simulink model "viikate_rocket"  (R2026b)
settings: Solver=ode4  StopTime=inf  FixedStep=0.001
undefined symbols (not defined in the file or in its folder): Aero, e0_0, e1_0, e2_0, e3_0, gravity, I, N, Newton, Raphson, rho, rp_burn_time_s, rp_canard_area_m2, rp_canard_cl_alpha, rp_cd0, rp_clp, rp_cmq, rp_cn_alpha, rp_cnr, rp_fin_positions_m, rp_frontal_area_m2, rp_gust_seed, rp_gust_variance, rp_ignition_time_s, rp_inertia_empty_kgm2, rp_inertia_full_kgm2, rp_length_m, rp_mass_fuel_kg, rp_mass_full_kg, rp_r_cp_m, rp_roll_ref_length_m, rp_servo_rate_limit_radps, rp_servo_tau_s, rp_thrust_n, rp_thrust_scale, rp_thrust_t_s, rp_wind_model_mps, sharedaeroassertmsg, si, Vsafe, ZYX
libraries: matrix_library x1
(part 2 of 3)

== system viikate_rocket/Simple Variable Mass 6DOF/Determine Force, Mass & Inertia/Estimate Inertia Tensor ==
  Mass : Inport
  M_dot : Inport  Port=2
  Constant : Constant  Value=emass
  Constant1 : Constant  Value=fmass
  "Interpolate Inertia " : Subsystem  mask(ScheduleMatrix-1D){matrix=I, aMode=aMode}
      mask prompts: matrix "shared_aeroblks:sharedaeroblkschedule:blockScheduleMatrix1DParamMatrixtointerpolate"
      mask help: shared_aeroblks:sharedaeroblkschedule:blockScheduleMatrix1DDesc
      mask init:
      | if aerosharedtest(gcb)
      |     aerosharedicon('shared');
      | else
      |     sharedautoicon('shared');
      | end
      mask Help: eval('if license(''test'',''Aerospace_Blockset'')aerosharedhelp(''interpolate_matrix_x'');elseif license(''test'',''Powertrain_Blockset'')sharedautohelp(''interpolate_matrix_x'');end')
      mask DialogControl matrix Prompt: Matrix to interpolate:
      mask Display:
      | port_label('input', 1,'x_k');
      | port_label('input', 2,'x_f');
      | port_label('output',1,'Matrix(x)');
  Mux : Mux  Inputs=2
  PreLook-Up Index Search : PreLookup  BreakpointsDataSource=Input port  BreakpointsData=[emass fmass]  BeginIndexSearchUsingPreviousIndexResult=on  IndexDataTypeStr=int32
      settings: InputPortMap=u0,p1
  Product : Product  SaturateOnIntegerOverflow=on  OutDataTypeStr=Inherit: Same as first input
  slope : Constant  Value=(fI - eI)/(fmass - emass)  OutDataTypeStr=Inherit: Inherit via back propagation
  Inertia : Outport  VectorParamsAs1DForOutWhenUnconnected=off
  I_dot : Outport  Port=2  VectorParamsAs1DForOutWhenUnconnected=off
  wires:
  "Interpolate Inertia "/1(Matrix(x)) -> Inertia/1
  Constant1/1 -> Mux/2
  Constant/1 -> Mux/1
  Mux/1 -> PreLook-Up Index Search/2
  PreLook-Up Index Search/1 -> "Interpolate Inertia "/1(x_k)
  PreLook-Up Index Search/2 -> "Interpolate Inertia "/2(x_f)
  Mass/1 -> PreLook-Up Index Search/1
  Product/1 -> I_dot/1
  M_dot/1 -> Product/2
  slope/1 -> Product/1

== system viikate_rocket/Simple Variable Mass 6DOF/Vbxw/Subsystem ==
  A : Inport
  B : Inport  Port=2
  Demux : Demux  Outputs=3
  Demux1 : Demux  Outputs=3
  Mux : Mux  Inputs=3
  i x j : Product  InputSameDT=on  SaturateOnIntegerOverflow=on  OutDataTypeStr=Inherit: Same as first input
  j x k : Product  InputSameDT=on  SaturateOnIntegerOverflow=on  OutDataTypeStr=Inherit: Same as first input
  k x i : Product  InputSameDT=on  SaturateOnIntegerOverflow=on  OutDataTypeStr=Inherit: Same as first input
  Out1 : Outport  VectorParamsAs1DForOutWhenUnconnected=off
  wires:
  Demux1/3 -> j x k/2
  Demux/2 -> j x k/1
  Demux/3 -> k x i/1
  Demux1/1 -> k x i/2
  Demux1/2 -> i x j/2
  Demux/1 -> i x j/1
  i x j/1 -> Mux/3
  k x i/1 -> Mux/2
  j x k/1 -> Mux/1
  B/1 -> Demux1/1
  A/1 -> Demux/1
  Mux/1 -> Out1/1

== system viikate_rocket/Simple Variable Mass 6DOF/Vbxw/Subsystem1 ==
  A : Inport
  B : Inport  Port=2
  Demux : Demux  Outputs=3
  Demux1 : Demux  Outputs=3
  Mux : Mux  Inputs=3
  i x k : Product  InputSameDT=on  SaturateOnIntegerOverflow=on  OutDataTypeStr=Inherit: Same as first input
  j x i : Product  InputSameDT=on  SaturateOnIntegerOverflow=on  OutDataTypeStr=Inherit: Same as first input
  k x j : Product  InputSameDT=on  SaturateOnIntegerOverflow=on  OutDataTypeStr=Inherit: Same as first input
  Out1 : Outport  VectorParamsAs1DForOutWhenUnconnected=off
  wires:
  j x i/1 -> Mux/3
  i x k/1 -> Mux/2
  k x j/1 -> Mux/1
  Mux/1 -> Out1/1
  Demux1/1 -> j x i/2
  Demux/2 -> j x i/1
  Demux1/3 -> i x k/2
  Demux/1 -> i x k/1
  Demux1/2 -> k x j/2
  Demux/3 -> k x j/1
  B/1 -> Demux1/1
  A/1 -> Demux/1

== system viikate_rocket/Simple Variable Mass 6DOF/Calculate DCM & Euler Angles/Quaternions to Direction Cosine Matrix/A11 ==
  normal(q) : Inport
  Demux : Demux
  Product{,1..3} (4 alike) : Product  RndMeth=Zero
  Sum : Sum  Inputs=++--
  A11 : Outport  VectorParamsAs1DForOutWhenUnconnected=off
  wires:
  Sum/1 -> A11/1
  Demux/4 -> Product/2, Product/1
  Demux/3 -> Product1/2, Product1/1
  Demux/2 -> Product2/2, Product2/1
  Demux/1 -> Product3/2, Product3/1
  Product3/1 -> Sum/1
  Product2/1 -> Sum/2
  Product1/1 -> Sum/3
  Product/1 -> Sum/4
  normal(q)/1 -> Demux/1

== system viikate_rocket/Simple Variable Mass 6DOF/Calculate DCM & Euler Angles/Quaternions to Direction Cosine Matrix/A12 ==
  normal(q) : Inport
  Demux : Demux
  Gain : Gain  Gain=2
  Product2 : Product  RndMeth=Zero
  Product3 : Product  RndMeth=Zero
  Sum : Sum  Inputs=|++
  A12 : Outport  VectorParamsAs1DForOutWhenUnconnected=off
  wires:
  Product2/1 -> Sum/2
  Product3/1 -> Sum/1
  Sum/1 -> Gain/1
  Demux/1 -> Product3/2
  Demux/2 -> Product2/1
  Demux/4 -> Product3/1
  Demux/3 -> Product2/2
  normal(q)/1 -> Demux/1
  Gain/1 -> A12/1

== system viikate_rocket/Simple Variable Mass 6DOF/Calculate DCM & Euler Angles/Quaternions to Direction Cosine Matrix/A13 ==
  normal(q) : Inport
  Demux : Demux
  Gain : Gain  Gain=2
  Product1 : Product  RndMeth=Zero
  Product2 : Product  RndMeth=Zero
  Sum : Sum  Inputs=|-+
  A13 : Outport  VectorParamsAs1DForOutWhenUnconnected=off
  wires:
  Demux/1 -> Product1/1
  Product1/1 -> Sum/1
  Product2/1 -> Sum/2
  Demux/4 -> Product2/2
  Demux/2 -> Product2/1
  Demux/3 -> Product1/2
  normal(q)/1 -> Demux/1
  Gain/1 -> A13/1
  Sum/1 -> Gain/1

== system viikate_rocket/Simple Variable Mass 6DOF/Calculate DCM & Euler Angles/Quaternions to Direction Cosine Matrix/A21 ==
  normal(q) : Inport
  Demux : Demux
  Gain : Gain  Gain=2
  Product2 : Product  RndMeth=Zero
  Product3 : Product  RndMeth=Zero
  Sum : Sum  Inputs=|-+
  A21 : Outport  VectorParamsAs1DForOutWhenUnconnected=off
  wires:
  Gain/1 -> A21/1
  normal(q)/1 -> Demux/1
  Demux/3 -> Product2/2
  Demux/4 -> Product3/1
  Demux/2 -> Product2/1
  Demux/1 -> Product3/2
  Sum/1 -> Gain/1
  Product3/1 -> Sum/1
  Product2/1 -> Sum/2

== system viikate_rocket/Simple Variable Mass 6DOF/Calculate DCM & Euler Angles/Quaternions to Direction Cosine Matrix/A22 ==
  normal(q) : Inport
  Demux : Demux
  Product{,1..3} (4 alike) : Product  RndMeth=Zero
  Sum : Sum  Inputs=+-+-
  A22 : Outport  VectorParamsAs1DForOutWhenUnconnected=off
  wires:
  normal(q)/1 -> Demux/1
  Product/1 -> Sum/4
  Product1/1 -> Sum/3
  Product2/1 -> Sum/2
  Product3/1 -> Sum/1
  Demux/1 -> Product3/1, Product3/2
  Demux/2 -> Product2/1, Product2/2
  Demux/3 -> Product1/1, Product1/2
  Demux/4 -> Product/1, Product/2
  Sum/1 -> A22/1

== system viikate_rocket/Simple Variable Mass 6DOF/Calculate DCM & Euler Angles/Quaternions to Direction Cosine Matrix/A23 ==
  normal(q) : Inport
  Demux : Demux
  Gain : Gain  Gain=2
  Product1 : Product  RndMeth=Zero
  Product2 : Product  RndMeth=Zero
  Sum : Sum  Inputs=|++
  A23 : Outport  VectorParamsAs1DForOutWhenUnconnected=off
  wires:
  Demux/4 -> Product2/2
  Product2/1 -> Sum/2
  Product1/1 -> Sum/1
  Sum/1 -> Gain/1
  Demux/1 -> Product1/1
  Demux/2 -> Product1/2
  Demux/3 -> Product2/1
  Gain/1 -> A23/1
  normal(q)/1 -> Demux/1

== system viikate_rocket/Simple Variable Mass 6DOF/Calculate DCM & Euler Angles/Quaternions to Direction Cosine Matrix/A31 ==
  normal(q) : Inport
  Demux : Demux
  Gain : Gain  Gain=2
  Product1 : Product  RndMeth=Zero
  Product2 : Product  RndMeth=Zero
  Sum : Sum  Inputs=|++
  A31 : Outport  VectorParamsAs1DForOutWhenUnconnected=off
  wires:
  Sum/1 -> Gain/1
  Gain/1 -> A31/1
  normal(q)/1 -> Demux/1
  Demux/3 -> Product1/2
  Demux/2 -> Product2/1
  Demux/4 -> Product2/2
  Product2/1 -> Sum/2
  Product1/1 -> Sum/1
  Demux/1 -> Product1/1

== system viikate_rocket/Simple Variable Mass 6DOF/Calculate DCM & Euler Angles/Quaternions to Direction Cosine Matrix/A32 ==
  normal(q) : Inport
  Demux : Demux
  Gain : Gain  Gain=2
  Product1 : Product  RndMeth=Zero
  Product2 : Product  RndMeth=Zero
  Sum : Sum  Inputs=|-+
  A32 : Outport  VectorParamsAs1DForOutWhenUnconnected=off
  wires:
  normal(q)/1 -> Demux/1
  Gain/1 -> A32/1
  Demux/3 -> Product2/1
  Demux/2 -> Product1/2
  Demux/1 -> Product1/1
  Sum/1 -> Gain/1
  Product1/1 -> Sum/1
  Product2/1 -> Sum/2
  Demux/4 -> Product2/2

== system viikate_rocket/Simple Variable Mass 6DOF/Calculate DCM & Euler Angles/Quaternions to Direction Cosine Matrix/A33 ==
  normal(q) : Inport
  Demux : Demux
  Product{,1..3} (4 alike) : Product  RndMeth=Zero
  Sum : Sum  Inputs=+--+
  A33 : Outport  VectorParamsAs1DForOutWhenUnconnected=off
  wires:
  normal(q)/1 -> Demux/1
  Product/1 -> Sum/4
  Product1/1 -> Sum/3
  Product2/1 -> Sum/2
  Product3/1 -> Sum/1
  Demux/1 -> Product3/1, Product3/2
  Demux/2 -> Product2/1, Product2/2
  Demux/3 -> Product1/1, Product1/2
  Demux/4 -> Product/1, Product/2
  Sum/1 -> A33/1

== system viikate_rocket/Simple Variable Mass 6DOF/Calculate DCM & Euler Angles/Quaternions to Direction Cosine Matrix/Create 3x3 Matrix ==
  M11 : Inport  PortDimensions=1
  M12 : Inport  Port=2  PortDimensions=1
  M13 : Inport  Port=3  PortDimensions=1
  M21 : Inport  Port=4  PortDimensions=1
  M22 : Inport  Port=5  PortDimensions=1
  M23 : Inport  Port=6  PortDimensions=1
  M31 : Inport  Port=7  PortDimensions=1
  M32 : Inport  Port=8  PortDimensions=1
  M33 : Inport  Port=9  PortDimensions=1
  Reshape (9) to [3x3] column-major : Reshape  OutputDimensionality=Customize  OutputDimensions=[3,3]
  Vector Concatenate : Concatenate  NumInputs=9
  Matrix : Outport  PortDimensions=[3 3]  VectorParamsAs1DForOutWhenUnconnected=off
  wires:
  M33/1 -> Vector Concatenate/9
  M23/1 -> Vector Concatenate/8
  M13/1 -> Vector Concatenate/7
  M32/1 -> Vector Concatenate/6
  Reshape (9) to [3x3] column-major/1 -> Matrix/1
  M22/1 -> Vector Concatenate/5
  M12/1 -> Vector Concatenate/4
  M31/1 -> Vector Concatenate/3
  M21/1 -> Vector Concatenate/2
  M11/1 -> Vector Concatenate/1
  Vector Concatenate/1 -> Reshape (9) to [3x3] column-major/1

== system viikate_rocket/Simple Variable Mass 6DOF/Calculate DCM & Euler Angles/Quaternions to Direction Cosine Matrix/Quaternion Normalize ==
  q : Inport  Unit=1
  Demux : Demux
  Mux : Mux
  Product{,1..3} (4 alike) : Product  Inputs=*/
  Quaternion Modulus : Subsystem  mask(Quaternion Modulus){aMode=aMode}
      mask help: shared_aeroblks:sharedaeroblkutil:blockQuaternionModulusDesc
      mask init:
      | if aerosharedtest(gcb)
      |     aerosharedicon('shared');
      | else
      |     sharedautoicon('shared');
      | end
      mask Help: eval('if license(''test'',''Aerospace_Blockset'')aerosharedhelp;elseif license(''test'',''Powertrain_Blockset'')sharedautohelp;end')
      mask Display:
      | port_label('input',  1, 'q')
      | port_label('output', 1, '|q|');
  normal(q) : Outport  Unit=1  VectorParamsAs1DForOutWhenUnconnected=off
  wires:
  Product3/1 -> Mux/4
  Product2/1 -> Mux/3
  Product1/1 -> Mux/2
  Product/1 -> Mux/1
  Quaternion Modulus/1(|q|) -> Product3/2, Product2/2, Product/2, Product1/2
  q/1 -> Demux/1, Quaternion Modulus/1(q)
  Mux/1 -> normal(q)/1
  Demux/1 -> Product/1
  Demux/2 -> Product1/1
  Demux/3 -> Product2/1
  Demux/4 -> Product3/1

== system viikate_rocket/Simple Variable Mass 6DOF/Calculate DCM & Euler Angles/Quaternions to Rotation Angles/DCM2Ang ==
  DCM : Inport  Unit=1
  AxisRotDefault : Subsystem  TreatAsAtomicUnit=on
  AxisRotZeroR3 : Subsystem  TreatAsAtomicUnit=on
  Get DCM Values : Subsystem
  If : If  IfExpression=(u1>=1)|(u1<=-1)
  Merge : Merge
  Selector4 : Selector  InputPortWidth=7  IndexOptions=Index vector (dialog)  Indices=3  OutputSizes=1  RuntimeRangeChecks=off
  Validate DCM : Subsystem  InitFcn=Aero.internal.maskutilities.validateDCMInit(gcb);  mask{action=action, tolerance=tolerance, aMode=aMode}
      mask prompts: action "shared_aeroblks:sharedaeroblktransform:action"; tolerance "shared_aeroblks:sharedaeroblktransform:actionTolerance"
      mask init:
      | if aerosharedtest(gcb) && builtin('license','test','Aerospace_Blockset')
      |     aerosharedicon('shared');
      | else
      |     sharedautoicon('shared');
      | end
      mask DialogControl action Prompt: Action for invalid DCM:
      mask DialogControl tolerance Prompt: Tolerance for DCM validation:
  Out1 : Outport  Unit=rad  VectorParamsAs1DForOutWhenUnconnected=off
  wires:
  AxisRotZeroR3/1(Out1) -> Merge/1
  AxisRotDefault/1(Out1) -> Merge/2
  If/1 -> AxisRotZeroR3/Action
  If/2 -> AxisRotDefault/Action
  Get DCM Values/1(Out1) -> AxisRotDefault/1(In1), AxisRotZeroR3/1(In1), Selector4/1
  Merge/1 -> Out1/1
  Selector4/1 -> If/1  "r21"
  DCM/1 -> Validate DCM/1(dcm), Get DCM Values/1(In1)

== system viikate_rocket/Simple Variable Mass 6DOF/Calculate DCM & Euler Angles/Quaternions to Rotation Angles/Quat2DCM ==
  Quat : Inport  Unit=1  PortDimensions=4
  A11 : Subsystem
  A12 : Subsystem
  A13 : Subsystem
  A21 : Subsystem
  A22 : Subsystem
  A23 : Subsystem
  A31 : Subsystem
  A32 : Subsystem
  A33 : Subsystem
  Create 3x3 Matrix : Subsystem  mask(Create 3x3 Matrix){aMode=aMode}
      mask help: shared_aeroblks:sharedaeroblkutil:blockCreate3x3MatrixDesc
      mask init:
      | if aerosharedtest(gcb)
      |     aerosharedicon('shared');
      | else
      |     sharedautoicon('shared');
      | end
      mask Help: eval('if license(''test'',''Aerospace_Blockset'')aerosharedhelp(''create_threebythree_matrix'');elseif license(''test'',''Powertrain_Blockset'')sharedautohelp(''create_threebythree_matrix'');end')
      mask Display:
      | port_label('input',1,'A_{11}','texmode','on');
      | port_label('input',2,'A_{12}','texmode','on');
      | port_label('input',3,'A_{13}','texmode','on');
      | port_label('input',4,'A_{21}','texmode','on');
      | port_label('input',5,'A_{22}','texmode','on');
      | port_label('input',6,'A_{23}','texmode','on');
      | port_label('input',7,'A_{31}','texmode','on');
      | port_label('input',8,'A_{32}','texmode','on');
      | port_label('input',9,'A_{33}','texmode','on');
      | port_label('output',1,'A','texmode','on');
  Quaternion Normalize : Subsystem  mask(Quaternion Normalize){aMode=aMode}
      mask help: shared_aeroblks:sharedaeroblkutil:blockQuaternionNormalizeDesc
      mask init:
      | if aerosharedtest(gcb)
      |     aerosharedicon('shared');
      | else
      |     sharedautoicon('shared');
      | end
      mask Help: eval('if license(''test'',''Aerospace_Blockset'')aerosharedhelp;elseif license(''test'',''Powertrain_Blockset'')sharedautohelp;end')
      mask Display:
      | port_label('input',  1, 'q')
      | port_label('output', 1, 'normal(q)');
  DCM : Outport  Unit=1  PortDimensions=[3,3]  InitialOutput=0  VectorParamsAs1DForOutWhenUnconnected=off
  wires:
  A11/1(A11) -> Create 3x3 Matrix/1(M11)
  A12/1(A12) -> Create 3x3 Matrix/2(M12)
  A13/1(A13) -> Create 3x3 Matrix/3(M13)
  A21/1(A21) -> Create 3x3 Matrix/4(M21)
  A22/1(A22) -> Create 3x3 Matrix/5(M22)
  A23/1(A23) -> Create 3x3 Matrix/6(M23)
  A31/1(A31) -> Create 3x3 Matrix/7(M31)
  A32/1(A32) -> Create 3x3 Matrix/8(M32)
  A33/1(A33) -> Create 3x3 Matrix/9(M33)
  Quaternion Normalize/1(normal(q)) -> A11/1(normal(q)), A12/1(normal(q)), A13/1(normal(q)), A21/1(normal(q)), A22/1(normal(q)), A23/1(normal(q)), A31/1(normal(q)), A32/1(normal(q)), A33/1(normal(q))
  Quat/1 -> Quaternion Normalize/1(q)
  Create 3x3 Matrix/1(Matrix) -> DCM/1

== system viikate_rocket/Simple Variable Mass 6DOF/Calculate omega_dot/3x3 Cross Product/Subsystem ==
  A : Inport
  B : Inport  Port=2
  Demux : Demux  Outputs=3
  Demux1 : Demux  Outputs=3
  Mux : Mux  Inputs=3
  i x j : Product  InputSameDT=on  SaturateOnIntegerOverflow=on  OutDataTypeStr=Inherit: Same as first input
  j x k : Product  InputSameDT=on  SaturateOnIntegerOverflow=on  OutDataTypeStr=Inherit: Same as first input
  k x i : Product  InputSameDT=on  SaturateOnIntegerOverflow=on  OutDataTypeStr=Inherit: Same as first input
  Out1 : Outport  VectorParamsAs1DForOutWhenUnconnected=off
  wires:
  Demux1/3 -> j x k/2
  Demux/2 -> j x k/1
  Demux/3 -> k x i/1
  Demux1/1 -> k x i/2
  Demux1/2 -> i x j/2
  Demux/1 -> i x j/1
  i x j/1 -> Mux/3
  k x i/1 -> Mux/2
  j x k/1 -> Mux/1
  B/1 -> Demux1/1
  A/1 -> Demux/1
  Mux/1 -> Out1/1

== system viikate_rocket/Simple Variable Mass 6DOF/Calculate omega_dot/3x3 Cross Product/Subsystem1 ==
  A : Inport
  B : Inport  Port=2
  Demux : Demux  Outputs=3
  Demux1 : Demux  Outputs=3
  Mux : Mux  Inputs=3
  i x k : Product  InputSameDT=on  SaturateOnIntegerOverflow=on  OutDataTypeStr=Inherit: Same as first input
  j x i : Product  InputSameDT=on  SaturateOnIntegerOverflow=on  OutDataTypeStr=Inherit: Same as first input
  k x j : Product  InputSameDT=on  SaturateOnIntegerOverflow=on  OutDataTypeStr=Inherit: Same as first input
  Out1 : Outport  VectorParamsAs1DForOutWhenUnconnected=off
  wires:
  j x i/1 -> Mux/3
  i x k/1 -> Mux/2
  k x j/1 -> Mux/1
  Mux/1 -> Out1/1
  Demux1/1 -> j x i/2
  Demux/2 -> j x i/1
  Demux1/3 -> i x k/2
  Demux/1 -> i x k/1
  Demux1/2 -> k x j/2
  Demux/3 -> k x j/1
  B/1 -> Demux1/1
  A/1 -> Demux/1

== system viikate_rocket/Simple Variable Mass 6DOF/Determine Force, Mass & Inertia/Estimate Inertia Tensor/Interpolate Inertia  ==
  x_k : Inport
  x_f : Inport  Port=2
  Matrix interpolation : Subsystem
  Matrix(x) : Outport  VectorParamsAs1DForOutWhenUnconnected=off
  wires:
  x_k/1 -> Matrix interpolation/1(index)
  x_f/1 -> Matrix interpolation/2(lambda_x)
  Matrix interpolation/1(matrix) -> Matrix(x)/1

== system viikate_rocket/Simple Variable Mass 6DOF/Calculate DCM & Euler Angles/Quaternions to Direction Cosine Matrix/Quaternion Normalize/Quaternion Modulus ==
  q : Inport  Unit=1
  Quaternion Norm : Subsystem  mask(Quaternion Norm){aMode=aMode}
      mask help: shared_aeroblks:sharedaeroblkutil:blockQuaternionNormDesc
      mask init:
      | if aerosharedtest(gcb)
      |     aerosharedicon('shared');
      | else
      |     sharedautoicon('shared');
      | end
      mask Help: eval('if license(''test'',''Aerospace_Blockset'')aerosharedhelp;elseif license(''test'',''Powertrain_Blockset'')sharedautohelp;end')
      mask Display:
      | port_label('input',  1, 'q');
      | port_label('output', 1, 'norm(q)');
  sqrt : Sqrt  RsqrtAlgorithmType=Newton-Raphson
  |q| : Outport  Unit=1  VectorParamsAs1DForOutWhenUnconnected=off
  wires:
  Quaternion Norm/1(norm(q)) -> sqrt/1
  q/1 -> Quaternion Norm/1(q)
  sqrt/1 -> |q|/1

== system viikate_rocket/Simple Variable Mass 6DOF/Calculate DCM & Euler Angles/Quaternions to Rotation Angles/DCM2Ang/AxisRotDefault ==
  In1 : Inport
  Action Port : ActionPort  ActionPortLabel=else
  Fcn1 : Fcn  Expr=atan2(u[1],u[2])
  Fcn2 : Fcn  Expr=asin(u)
  Fcn3 : Fcn  Expr=atan2(u[4],u[5])
  Protect asincos input : Subsystem  mask{aMode=aMode}
      mask init:
      | if aerosharedtest(gcb) && builtin('license','test','Aerospace_Blockset')
      |     aerosharedicon('shared');
      | else
      |     sharedautoicon('shared');
      | end
  Selector : Selector  InputPortWidth=7  IndexOptions=Index vector (dialog)  Indices=3  OutputSizes=1  RuntimeRangeChecks=off
  Vector Concatenate : Concatenate  NumInputs=3
  Out1 : Outport  VectorParamsAs1DForOutWhenUnconnected=off
  wires:
  Vector Concatenate/1 -> Out1/1
  Fcn3/1 -> Vector Concatenate/3  "r3"
  Fcn2/1 -> Vector Concatenate/2  "r2"
  Fcn1/1 -> Vector Concatenate/1  "r1"
  In1/1 -> Selector/1, Fcn1/1, Fcn3/1
  Protect asincos input/1(Out) -> Fcn2/1
  Selector/1 -> Protect asincos input/1(In)

== system viikate_rocket/Simple Variable Mass 6DOF/Calculate DCM & Euler Angles/Quaternions to Rotation Angles/DCM2Ang/AxisRotZeroR3 ==
  In1 : Inport
  Action Port : ActionPort  ActionPortLabel=if((u1>=1)|(u1<=-1))
  Fcn1 : Fcn  Expr=atan2(u[6],u[7])
  Fcn2 : Fcn  Expr=asin(u)
  Fcn3 : Fcn  Expr=0
  Protect asincos input : Subsystem  mask{aMode=aMode}
      mask init:
      | if aerosharedtest(gcb) && builtin('license','test','Aerospace_Blockset')
      |     aerosharedicon('shared');
      | else
      |     sharedautoicon('shared');
      | end
  Selector : Selector  InputPortWidth=7  IndexOptions=Index vector (dialog)  Indices=3  OutputSizes=1  RuntimeRangeChecks=off
  Vector Concatenate : Concatenate  NumInputs=3
  Out1 : Outport  VectorParamsAs1DForOutWhenUnconnected=off
  wires:
  In1/1 -> Selector/1, Fcn1/1, Fcn3/1
  Fcn1/1 -> Vector Concatenate/1  "r1"
  Fcn2/1 -> Vector Concatenate/2  "r2"
  Fcn3/1 -> Vector Concatenate/3  "r3"
  Vector Concatenate/1 -> Out1/1
  Protect asincos input/1(Out) -> Fcn2/1
  Selector/1 -> Protect asincos input/1(In)

== system viikate_rocket/Simple Variable Mass 6DOF/Calculate DCM & Euler Angles/Quaternions to Rotation Angles/DCM2Ang/Get DCM Values ==
  In1 : Inport
  Gain1 : Gain  Gain=[1 1 -1]
  Gain2 : Gain  Gain=[1 1]
  Gain3 : Gain  Gain=[-1 1]
  Reshape : Reshape
  Reshape1 : Reshape
  Reshape2 : Reshape
  Selector1 : Selector  NumberOfDimensions=2  InputPortWidth=3  IndexOptions=Index vector (dialog),Index vector (dialog)  Indices=1,[2 1 3]  OutputSizes=1,1  RuntimeRangeChecks=off
  Selector2 : Selector  NumberOfDimensions=2  InputPortWidth=3  IndexOptions=Index vector (dialog),Index vector (dialog)  Indices=[2 3],3  OutputSizes=1,1  RuntimeRangeChecks=off
  Selector3 : Selector  NumberOfDimensions=2  InputPortWidth=3  IndexOptions=Index vector (dialog),Index vector (dialog)  Indices=2,[1 2]  OutputSizes=1,1  RuntimeRangeChecks=off
  Vector Concatenate : Concatenate  NumInputs=3
  Out1 : Outport  VectorParamsAs1DForOutWhenUnconnected=off
  wires:
  Vector Concatenate/1 -> Out1/1
  Gain3/1 -> Vector Concatenate/3
  Gain2/1 -> Vector Concatenate/2
  Gain1/1 -> Vector Concatenate/1
  In1/1 -> Selector3/1, Selector2/1, Selector1/1
  Reshape2/1 -> Gain3/1
  Reshape1/1 -> Gain2/1
  Reshape/1 -> Gain1/1
  Selector1/1 -> Reshape/1
  Selector2/1 -> Reshape1/1
  Selector3/1 -> Reshape2/1

== system viikate_rocket/Simple Variable Mass 6DOF/Calculate DCM & Euler Angles/Quaternions to Rotation Angles/DCM2Ang/Validate DCM ==
  note: action can be: None (1), Warning (2), or Error (3)
  dcm : Inport
  Constant : Constant  Value=action  OutDataTypeStr=uint8
  If Warning/Error : Subsystem  TreatAsAtomicUnit=on
  If1 : If  IfExpression=u1 > 1  ShowElse=off
  wires:
  If1/1 -> If Warning/Error/Action
  dcm/1 -> If Warning/Error/1(dcm)
  Constant/1 -> If1/1

== system viikate_rocket/Simple Variable Mass 6DOF/Calculate DCM & Euler Angles/Quaternions to Rotation Angles/Quat2DCM/A11 ==
  normal(q) : Inport
  Demux : Demux
  Product{,1..3} (4 alike) : Product  RndMeth=Zero
  Sum : Sum  Inputs=++--
  A11 : Outport  VectorParamsAs1DForOutWhenUnconnected=off
  wires:
  Sum/1 -> A11/1
  Demux/4 -> Product/2, Product/1
  Demux/3 -> Product1/2, Product1/1
  Demux/2 -> Product2/2, Product2/1
  Demux/1 -> Product3/2, Product3/1
  Product3/1 -> Sum/1
  Product2/1 -> Sum/2
  Product1/1 -> Sum/3
  Product/1 -> Sum/4
  normal(q)/1 -> Demux/1

== system viikate_rocket/Simple Variable Mass 6DOF/Calculate DCM & Euler Angles/Quaternions to Rotation Angles/Quat2DCM/A12 ==
  normal(q) : Inport
  Demux : Demux
  Gain : Gain  Gain=2
  Product2 : Product  RndMeth=Zero
  Product3 : Product  RndMeth=Zero
  Sum : Sum  Inputs=|++
  A12 : Outport  VectorParamsAs1DForOutWhenUnconnected=off
  wires:
  Product2/1 -> Sum/2
  Product3/1 -> Sum/1
  Sum/1 -> Gain/1
  Demux/1 -> Product3/2
  Demux/2 -> Product2/1
  Demux/4 -> Product3/1
  Demux/3 -> Product2/2
  normal(q)/1 -> Demux/1
  Gain/1 -> A12/1

== system viikate_rocket/Simple Variable Mass 6DOF/Calculate DCM & Euler Angles/Quaternions to Rotation Angles/Quat2DCM/A13 ==
  normal(q) : Inport
  Demux : Demux
  Gain : Gain  Gain=2
  Product1 : Product  RndMeth=Zero
  Product2 : Product  RndMeth=Zero
  Sum : Sum  Inputs=|-+
  A13 : Outport  VectorParamsAs1DForOutWhenUnconnected=off
  wires:
  Demux/1 -> Product1/1
  Product1/1 -> Sum/1
  Product2/1 -> Sum/2
  Demux/4 -> Product2/2
  Demux/2 -> Product2/1
  Demux/3 -> Product1/2
  normal(q)/1 -> Demux/1
  Gain/1 -> A13/1
  Sum/1 -> Gain/1

== system viikate_rocket/Simple Variable Mass 6DOF/Calculate DCM & Euler Angles/Quaternions to Rotation Angles/Quat2DCM/A21 ==
  normal(q) : Inport
  Demux : Demux
  Gain : Gain  Gain=2
  Product2 : Product  RndMeth=Zero
  Product3 : Product  RndMeth=Zero
  Sum : Sum  Inputs=|-+
  A21 : Outport  VectorParamsAs1DForOutWhenUnconnected=off
  wires:
  Gain/1 -> A21/1
  normal(q)/1 -> Demux/1
  Demux/3 -> Product2/2
  Demux/4 -> Product3/1
  Demux/2 -> Product2/1
  Demux/1 -> Product3/2
  Sum/1 -> Gain/1
  Product3/1 -> Sum/1
  Product2/1 -> Sum/2

== system viikate_rocket/Simple Variable Mass 6DOF/Calculate DCM & Euler Angles/Quaternions to Rotation Angles/Quat2DCM/A22 ==
  normal(q) : Inport
  Demux : Demux
  Product{,1..3} (4 alike) : Product  RndMeth=Zero
  Sum : Sum  Inputs=+-+-
  A22 : Outport  VectorParamsAs1DForOutWhenUnconnected=off
  wires:
  normal(q)/1 -> Demux/1
  Product/1 -> Sum/4
  Product1/1 -> Sum/3
  Product2/1 -> Sum/2
  Product3/1 -> Sum/1
  Demux/1 -> Product3/1, Product3/2
  Demux/2 -> Product2/1, Product2/2
  Demux/3 -> Product1/1, Product1/2
  Demux/4 -> Product/1, Product/2
  Sum/1 -> A22/1

== system viikate_rocket/Simple Variable Mass 6DOF/Calculate DCM & Euler Angles/Quaternions to Rotation Angles/Quat2DCM/A23 ==
  normal(q) : Inport
  Demux : Demux
  Gain : Gain  Gain=2
  Product1 : Product  RndMeth=Zero
  Product2 : Product  RndMeth=Zero
  Sum : Sum  Inputs=|++
  A23 : Outport  VectorParamsAs1DForOutWhenUnconnected=off
  wires:
  Demux/4 -> Product2/2
  Product2/1 -> Sum/2
  Product1/1 -> Sum/1
  Sum/1 -> Gain/1
  Demux/1 -> Product1/1
  Demux/2 -> Product1/2
  Demux/3 -> Product2/1
  Gain/1 -> A23/1
  normal(q)/1 -> Demux/1

== system viikate_rocket/Simple Variable Mass 6DOF/Calculate DCM & Euler Angles/Quaternions to Rotation Angles/Quat2DCM/A31 ==
  normal(q) : Inport
  Demux : Demux
  Gain : Gain  Gain=2
  Product1 : Product  RndMeth=Zero
  Product2 : Product  RndMeth=Zero
  Sum : Sum  Inputs=|++
  A31 : Outport  VectorParamsAs1DForOutWhenUnconnected=off
  wires:
  Sum/1 -> Gain/1
  Gain/1 -> A31/1
  normal(q)/1 -> Demux/1
  Demux/3 -> Product1/2
  Demux/2 -> Product2/1
  Demux/4 -> Product2/2
  Product2/1 -> Sum/2
  Product1/1 -> Sum/1
  Demux/1 -> Product1/1

== system viikate_rocket/Simple Variable Mass 6DOF/Calculate DCM & Euler Angles/Quaternions to Rotation Angles/Quat2DCM/A32 ==
  normal(q) : Inport
  Demux : Demux
  Gain : Gain  Gain=2
  Product1 : Product  RndMeth=Zero
  Product2 : Product  RndMeth=Zero
  Sum : Sum  Inputs=|-+
  A32 : Outport  VectorParamsAs1DForOutWhenUnconnected=off
  wires:
  normal(q)/1 -> Demux/1
  Gain/1 -> A32/1
  Demux/3 -> Product2/1
  Demux/2 -> Product1/2
  Demux/1 -> Product1/1
  Sum/1 -> Gain/1
  Product1/1 -> Sum/1
  Product2/1 -> Sum/2
  Demux/4 -> Product2/2

== system viikate_rocket/Simple Variable Mass 6DOF/Calculate DCM & Euler Angles/Quaternions to Rotation Angles/Quat2DCM/A33 ==
  normal(q) : Inport
  Demux : Demux
  Product{,1..3} (4 alike) : Product  RndMeth=Zero
  Sum : Sum  Inputs=+--+
  A33 : Outport  VectorParamsAs1DForOutWhenUnconnected=off
  wires:
  normal(q)/1 -> Demux/1
  Product/1 -> Sum/4
  Product1/1 -> Sum/3
  Product2/1 -> Sum/2
  Product3/1 -> Sum/1
  Demux/1 -> Product3/1, Product3/2
  Demux/2 -> Product2/1, Product2/2
  Demux/3 -> Product1/1, Product1/2
  Demux/4 -> Product/1, Product/2
  Sum/1 -> A33/1

== system viikate_rocket/Simple Variable Mass 6DOF/Calculate DCM & Euler Angles/Quaternions to Rotation Angles/Quat2DCM/Create 3x3 Matrix ==
  M11 : Inport  PortDimensions=1
  M12 : Inport  Port=2  PortDimensions=1
  M13 : Inport  Port=3  PortDimensions=1
  M21 : Inport  Port=4  PortDimensions=1
  M22 : Inport  Port=5  PortDimensions=1
  M23 : Inport  Port=6  PortDimensions=1
  M31 : Inport  Port=7  PortDimensions=1
  M32 : Inport  Port=8  PortDimensions=1
  M33 : Inport  Port=9  PortDimensions=1
  Reshape (9) to [3x3] column-major : Reshape  OutputDimensionality=Customize  OutputDimensions=[3,3]
  Vector Concatenate : Concatenate  NumInputs=9
  Matrix : Outport  PortDimensions=[3 3]  VectorParamsAs1DForOutWhenUnconnected=off
  wires:
  M33/1 -> Vector Concatenate/9
  M23/1 -> Vector Concatenate/8
  M13/1 -> Vector Concatenate/7
  M32/1 -> Vector Concatenate/6
  Reshape (9) to [3x3] column-major/1 -> Matrix/1
  M22/1 -> Vector Concatenate/5
  M12/1 -> Vector Concatenate/4
  M31/1 -> Vector Concatenate/3
  M21/1 -> Vector Concatenate/2
  M11/1 -> Vector Concatenate/1
  Vector Concatenate/1 -> Reshape (9) to [3x3] column-major/1

== system viikate_rocket/Simple Variable Mass 6DOF/Calculate DCM & Euler Angles/Quaternions to Rotation Angles/Quat2DCM/Quaternion Normalize ==
  q : Inport  Unit=1
  Demux : Demux
  Mux : Mux
  Product{,1..3} (4 alike) : Product  Inputs=*/
  Quaternion Modulus : Subsystem  mask(Quaternion Modulus){aMode=aMode}
      mask help: shared_aeroblks:sharedaeroblkutil:blockQuaternionModulusDesc
      mask init:
      | if aerosharedtest(gcb)
      |     aerosharedicon('shared');
      | else
      |     sharedautoicon('shared');
      | end
      mask Help: eval('if license(''test'',''Aerospace_Blockset'')aerosharedhelp;elseif license(''test'',''Powertrain_Blockset'')sharedautohelp;end')
      mask Display:
      | port_label('input',  1, 'q')
      | port_label('output', 1, '|q|');
  normal(q) : Outport  Unit=1  VectorParamsAs1DForOutWhenUnconnected=off
  wires:
  Product3/1 -> Mux/4
  Product2/1 -> Mux/3
  Product1/1 -> Mux/2
  Product/1 -> Mux/1
  Quaternion Modulus/1(|q|) -> Product3/2, Product2/2, Product/2, Product1/2
  q/1 -> Demux/1, Quaternion Modulus/1(q)
  Mux/1 -> normal(q)/1
  Demux/1 -> Product/1
  Demux/2 -> Product1/1
  Demux/3 -> Product2/1
  Demux/4 -> Product3/1

== system viikate_rocket/Simple Variable Mass 6DOF/Determine Force, Mass & Inertia/Estimate Inertia Tensor/Interpolate Inertia /Matrix interpolation ==
  index : Inport
  lambda_x : Inport  Port=2  PortDimensions=1
  1-lambda_x : Product  SaturateOnIntegerOverflow=on  OutDataTypeStr=Inherit: Same as first input
  Fcn : Fcn  Expr=1-u(1)
  Sum : Sum  Inputs=|++  InputSameDT=on  SaturateOnIntegerOverflow=on  OutDataTypeStr=Inherit: Same as first input
  Sum3 : Sum  Inputs=+|+  OutDataTypeStr=Inherit: Inherit via back propagation  SaturateOnIntegerOverflow=on
  Terminator_Sum : Terminator
  "[0]" : Constant  Value=rp_inertia_empty_kgm2
  "[1]" : Constant  Value=rp_inertia_full_kgm2
  lambda_x. : Product  SaturateOnIntegerOverflow=on  OutDataTypeStr=Inherit: Same as first input
  offset for upper index 1 : Constant  OutDataTypeStr=Inherit: Inherit via back propagation
  matrix : Outport  VectorParamsAs1DForOutWhenUnconnected=off
  wires:
  lambda_x/1 -> Fcn/1, lambda_x./2
  index/1 -> Sum/1
  offset for upper index 1/1 -> Sum/2
  Fcn/1 -> 1-lambda_x/2
  1-lambda_x/1 -> Sum3/1
  lambda_x./1 -> Sum3/2
  Sum3/1 -> matrix/1
  "[0]"/1 -> 1-lambda_x/1
  "[1]"/1 -> lambda_x./1
  Sum/1 -> Terminator_Sum/1

== system viikate_rocket/Simple Variable Mass 6DOF/Calculate DCM & Euler Angles/Quaternions to Direction Cosine Matrix/Quaternion Normalize/Quaternion Modulus/Quaternion Norm ==
  q : Inport  Unit=1
  Demux : Demux
  Product{,1..3} (4 alike) : Product
  Sum : Sum  Inputs=4
  norm(q) : Outport  Unit=1  VectorParamsAs1DForOutWhenUnconnected=off
  wires:
  Demux/4 -> Product3/1, Product3/2
  Demux/3 -> Product2/1, Product2/2
  Demux/2 -> Product1/1, Product1/2
  Demux/1 -> Product/1, Product/2
  Product3/1 -> Sum/4
  Product2/1 -> Sum/3
  Product1/1 -> Sum/2
  Product/1 -> Sum/1
  Sum/1 -> norm(q)/1
  q/1 -> Demux/1

== system viikate_rocket/Simple Variable Mass 6DOF/Calculate DCM & Euler Angles/Quaternions to Rotation Angles/DCM2Ang/AxisRotDefault/Protect asincos input ==
  In : Inport
  If : If  IfExpression=u1 > 1  ElseIfExpressions=u1 < -1
  If Action Subsystem : Subsystem  TreatAsAtomicUnit=on
  If Action Subsystem1 : Subsystem  TreatAsAtomicUnit=on
  If Action Subsystem2 : Subsystem  TreatAsAtomicUnit=on
  Merge : Merge  Inputs=3
  Out : Outport  VectorParamsAs1DForOutWhenUnconnected=off
  wires:
  Merge/1 -> Out/1
  If Action Subsystem2/1(OutOrig) -> Merge/3
  If Action Subsystem1/1(OutputNeg1) -> Merge/2
  If Action Subsystem/1(OutputPos1) -> Merge/1
  If/3 -> If Action Subsystem2/Action
  If/2 -> If Action Subsystem1/Action
  In/1 -> If/1, If Action Subsystem2/1(In)
  If/1 -> If Action Subsystem/Action

== system viikate_rocket/Simple Variable Mass 6DOF/Calculate DCM & Euler Angles/Quaternions to Rotation Angles/DCM2Ang/AxisRotZeroR3/Protect asincos input ==
  In : Inport
  If : If  IfExpression=u1 > 1  ElseIfExpressions=u1 < -1
  If Action Subsystem : Subsystem  TreatAsAtomicUnit=on
  If Action Subsystem1 : Subsystem  TreatAsAtomicUnit=on
  If Action Subsystem2 : Subsystem  TreatAsAtomicUnit=on
  Merge : Merge  Inputs=3
  Out : Outport  VectorParamsAs1DForOutWhenUnconnected=off
  wires:
  Merge/1 -> Out/1
  If Action Subsystem2/1(OutOrig) -> Merge/3
  If Action Subsystem1/1(OutputNeg1) -> Merge/2
  If Action Subsystem/1(OutputPos1) -> Merge/1
  If/3 -> If Action Subsystem2/Action
  If/2 -> If Action Subsystem1/Action
  In/1 -> If/1, If Action Subsystem2/1(In)
  If/1 -> If Action Subsystem/Action

== system viikate_rocket/Simple Variable Mass 6DOF/Calculate DCM & Euler Angles/Quaternions to Rotation Angles/DCM2Ang/Validate DCM/If Warning//Error ==
  dcm : Inport
  if : ActionPort  InitializeStates=reset  ActionPortLabel=if(u1 > 1)
  Else If Not Orthogonal : Subsystem  TreatAsAtomicUnit=on
  Else No Action : Subsystem  TreatAsAtomicUnit=on
  If : If  NumInputs=2  IfExpression=u1 == 1  ElseIfExpressions=u2 == 1
  If Not Proper : Subsystem  TreatAsAtomicUnit=on
  Verify Size : SignalSpecification  Dimensions=[3,3]
  isNotOrthogonal : Subsystem
  isNotProper : Subsystem
  wires:
  If/3 -> Else No Action/Action
  If/2 -> Else If Not Orthogonal/Action
  If/1 -> If Not Proper/Action
  isNotOrthogonal/1(Out) -> If/2
  isNotProper/1(Out) -> If/1
  Verify Size/1 -> isNotProper/1(dcm), isNotOrthogonal/1(dcm)
  dcm/1 -> Verify Size/1

== system viikate_rocket/Simple Variable Mass 6DOF/Calculate DCM & Euler Angles/Quaternions to Rotation Angles/Quat2DCM/Quaternion Normalize/Quaternion Modulus ==
  q : Inport  Unit=1
  Quaternion Norm : Subsystem  mask(Quaternion Norm){aMode=aMode}
      mask help: shared_aeroblks:sharedaeroblkutil:blockQuaternionNormDesc
      mask init:
      | if aerosharedtest(gcb)
      |     aerosharedicon('shared');
      | else
      |     sharedautoicon('shared');
      | end
      mask Help: eval('if license(''test'',''Aerospace_Blockset'')aerosharedhelp;elseif license(''test'',''Powertrain_Blockset'')sharedautohelp;end')
      mask Display:
      | port_label('input',  1, 'q');
      | port_label('output', 1, 'norm(q)');
  sqrt : Sqrt  RsqrtAlgorithmType=Newton-Raphson
  |q| : Outport  Unit=1  VectorParamsAs1DForOutWhenUnconnected=off
  wires:
  Quaternion Norm/1(norm(q)) -> sqrt/1
  q/1 -> Quaternion Norm/1(q)
  sqrt/1 -> |q|/1

== system viikate_rocket/Simple Variable Mass 6DOF/Calculate DCM & Euler Angles/Quaternions to Rotation Angles/DCM2Ang/AxisRotDefault/Protect asincos input/If Action Subsystem ==
  Action Port : ActionPort  ActionPortLabel=if(u1 > 1)
  Constant : Constant  OutDataTypeStr=Inherit: Inherit via back propagation  SampleTime=-1
  OutputPos1 : Outport  InitialOutput=0  VectorParamsAs1DForOutWhenUnconnected=off
  wires:
  Constant/1 -> OutputPos1/1

== system viikate_rocket/Simple Variable Mass 6DOF/Calculate DCM & Euler Angles/Quaternions to Rotation Angles/DCM2Ang/AxisRotDefault/Protect asincos input/If Action Subsystem1 ==
  Action Port : ActionPort  ActionPortLabel=elseif(u1 < -1)
  Constant : Constant  Value=-1  OutDataTypeStr=Inherit: Inherit via back propagation  SampleTime=-1
  OutputNeg1 : Outport  InitialOutput=0  VectorParamsAs1DForOutWhenUnconnected=off
  wires:
  Constant/1 -> OutputNeg1/1

== system viikate_rocket/Simple Variable Mass 6DOF/Calculate DCM & Euler Angles/Quaternions to Rotation Angles/DCM2Ang/AxisRotDefault/Protect asincos input/If Action Subsystem2 ==
  In : Inport
  Action Port : ActionPort  ActionPortLabel=else
  OutOrig : Outport  InitialOutput=0  VectorParamsAs1DForOutWhenUnconnected=off
  wires:
  In/1 -> OutOrig/1

== system viikate_rocket/Simple Variable Mass 6DOF/Calculate DCM & Euler Angles/Quaternions to Rotation Angles/DCM2Ang/AxisRotZeroR3/Protect asincos input/If Action Subsystem ==
  Action Port : ActionPort  ActionPortLabel=if(u1 > 1)
  Constant : Constant  OutDataTypeStr=Inherit: Inherit via back propagation  SampleTime=-1
  OutputPos1 : Outport  InitialOutput=0  VectorParamsAs1DForOutWhenUnconnected=off
  wires:
  Constant/1 -> OutputPos1/1

== system viikate_rocket/Simple Variable Mass 6DOF/Calculate DCM & Euler Angles/Quaternions to Rotation Angles/DCM2Ang/AxisRotZeroR3/Protect asincos input/If Action Subsystem1 ==
  Action Port : ActionPort  ActionPortLabel=elseif(u1 < -1)
  Constant : Constant  Value=-1  OutDataTypeStr=Inherit: Inherit via back propagation  SampleTime=-1
  OutputNeg1 : Outport  InitialOutput=0  VectorParamsAs1DForOutWhenUnconnected=off
  wires:
  Constant/1 -> OutputNeg1/1

== system viikate_rocket/Simple Variable Mass 6DOF/Calculate DCM & Euler Angles/Quaternions to Rotation Angles/DCM2Ang/AxisRotZeroR3/Protect asincos input/If Action Subsystem2 ==
  In : Inport
  Action Port : ActionPort  ActionPortLabel=else
  OutOrig : Outport  InitialOutput=0  VectorParamsAs1DForOutWhenUnconnected=off
  wires:
  In/1 -> OutOrig/1

== system viikate_rocket/Simple Variable Mass 6DOF/Calculate DCM & Euler Angles/Quaternions to Rotation Angles/DCM2Ang/Validate DCM/If Warning//Error/Else If Not Orthogonal ==
  Action Port : ActionPort  InitializeStates=reset  ActionPortLabel=elseif(u2 == 1)
  Constant : Constant  Value=action  OutDataTypeStr=uint8
  Constant1 : Constant  Value=0
  Error : Subsystem  TreatAsAtomicUnit=on
  If : If  IfExpression=u1 == 2  ElseIfExpressions=u1 == 3
  None : Subsystem  TreatAsAtomicUnit=on
  Warning : Subsystem  TreatAsAtomicUnit=on
  wires:
  If/3 -> None/Action
  If/2 -> Error/Action
  If/1 -> Warning/Action
  Constant/1 -> If/1
  Constant1/1 -> Warning/1(In), Error/1(In)

== system viikate_rocket/Simple Variable Mass 6DOF/Calculate DCM & Euler Angles/Quaternions to Rotation Angles/DCM2Ang/Validate DCM/If Warning//Error/Else No Action ==
  Action Port : ActionPort  ActionPortLabel=else

== system viikate_rocket/Simple Variable Mass 6DOF/Calculate DCM & Euler Angles/Quaternions to Rotation Angles/DCM2Ang/Validate DCM/If Warning//Error/If Not Proper ==
  Action Port : ActionPort  ActionPortLabel=if(u1 == 1)
  Constant : Constant  Value=action  OutDataTypeStr=uint8
  Constant1 : Constant  Value=0
  Error : Subsystem  TreatAsAtomicUnit=on
  If : If  IfExpression=u1 == 2  ElseIfExpressions=u1 == 3
  None : Subsystem  TreatAsAtomicUnit=on
  Warning : Subsystem  TreatAsAtomicUnit=on
  wires:
  If/3 -> None/Action
  Constant1/1 -> Warning/1(In), Error/1(In)
  Constant/1 -> If/1
  If/1 -> Warning/Action
  If/2 -> Error/Action

== system viikate_rocket/Simple Variable Mass 6DOF/Calculate DCM & Euler Angles/Quaternions to Rotation Angles/DCM2Ang/Validate DCM/If Warning//Error/isNotOrthogonal ==
  dcm : Inport
  Abs2 : Abs  SaturateOnIntegerOverflow=off
  Bias1 : Bias  Bias=-eye(3)  SaturateOnIntegerOverflow=off
  Logical Operator1 : Logic  Operator=OR  Inputs=1  AllPortsSameDT=off  OutDataTypeStr=boolean
  Math Function : Math  Operator=transpose  SignedPower=on
  Product : Product  Multiplication=Matrix(*)
  Reshape : Reshape  OutputDimensionality=Column vector (2-D)  OutputDimensions=[9,1]
  transpose*dcm ~= eye(3) : Subsystem  mask(Compare To Constant){relop=>, const=tolerance, OutDataTypeStr=boolean, ZeroCross=on}
      mask prompts: relop "Simulink:masks:Operator_MP"; const "Simulink:masks:ConstantValue_MP"; OutDataTypeStr "Simulink:masks:OutputDataType_MP"; ZeroCross "Simulink:masks:EnableZerocrossingDetection_MP"
      mask help: Simulink:masks:CompareToConstant_MD
      mask init:
      | blkName = gcb;
      | 
      | if strcmp(get_param(gcbh,'OutDataTypeStr'),'boolean')
      | 	setValue = 'boolean';
      | else
      | 	setValue = 'fixdt(0, 8, 0)';
      | end
      | 
      | set_param([blkName,'/Compare'],'relop',relop, ...
      | 	'OutDataTypeStr', setValue, 'ZeroCross', ZeroCross);
      | 
      | str = [relop,' C']; %default
      | 
      | const_str = get_param(blkName, 'const');
      | const_val = str2num(const_str, 'Evaluation','restricted');
      | 
      | if isempty(const_val) %#ok<ST2NM>
      |     %Expression/Variable
      |     str = [relop, ' ', strtrim(const_str)];
      | else
      |     if length(const_val) == 1 
      |         if Simulink.data.isSupportedEnumClass(class(const_val))
      |             % Special Handling for Enumerations
      |             if Simulink.data.getEnumTypeInfo(class(const_val), 'AddClassNameToEnumNames')
      |                 str = [relop, ' ', strtrim(const_str)];
      |             else
      |                 str = [relop, ' ', char(const_val)];
      |             end
      |         elseif(isfloat(const_val) || isinteger(const_val) || islogical(const_val)) 
      |                 str = [relop, ' ', num2str(const_val)];
      |         end
      |     end
      | end
      mask TypeOptions relop: == | ~= | < | <= | >= | >
      mask TypeOptions OutDataTypeStr: Simulink:masks:uint8 | Simulink:masks:boolean
      mask Callback ZeroCross: sl('zeroCrossEnable', gcbh);
      mask Display: disp(str)
  Out : Outport  VectorParamsAs1DForOutWhenUnconnected=off
  wires:
  Reshape/1 -> Logical Operator1/1
  Product/1 -> Bias1/1
  transpose*dcm ~= eye(3)/1(y) -> Reshape/1
  Abs2/1 -> transpose*dcm ~= eye(3)/1(u)
  Bias1/1 -> Abs2/1
  dcm/1 -> Math Function/1, Product/2
  Math Function/1 -> Product/1
  Logical Operator1/1 -> Out/1

== system viikate_rocket/Simple Variable Mass 6DOF/Calculate DCM & Euler Angles/Quaternions to Rotation Angles/DCM2Ang/Validate DCM/If Warning//Error/isNotProper ==
  dcm : Inport
  Abs1 : Abs  SaturateOnIntegerOverflow=off
  Bias : Bias  Bias=-1  SaturateOnIntegerOverflow=off
  Determinant of 3x3 Matrix : Subsystem  mask(Determinant of 3x3 Matrix){aMode=aMode}
      mask help: shared_aeroblks:sharedaeroblkutil:blockDeterminantof3x3MatrixDesc
      mask init:
      | if aerosharedtest(gcb)
      |     aerosharedicon('shared');
      | else
      |     sharedautoicon('shared');
      | end
      mask Help: eval('if license(''test'',''Aerospace_Blockset'')aerosharedhelp(''determinant_of_3by3_matrix'');elseif license(''test'',''Powertrain_Blockset'')sharedautohelp(''determinant_of_3by3_matrix'');end')
      mask Display:
      | text(.5,.5,'det(A)\n(3x3)',...
      | 	'horizontalalignment','center');
  determinant does not equal 1 : Subsystem  mask(Compare To Constant){relop=>, const=tolerance, OutDataTypeStr=boolean, ZeroCross=on}
      mask prompts: relop "Simulink:masks:Operator_MP"; const "Simulink:masks:ConstantValue_MP"; OutDataTypeStr "Simulink:masks:OutputDataType_MP"; ZeroCross "Simulink:masks:EnableZerocrossingDetection_MP"
      mask help: Simulink:masks:CompareToConstant_MD
      mask init: same as viikate_rocket/Simple Variable Mass 6DOF/Calculate DCM & Euler Angles/Quaternions to Rotation Angles/DCM2Ang/Validate DCM/If Warning//Error/isNotOrthogonal/transpose*dcm ~= eye(3)
      mask TypeOptions relop: == | ~= | < | <= | >= | >
      mask TypeOptions OutDataTypeStr: Simulink:masks:uint8 | Simulink:masks:boolean
      mask Callback ZeroCross: sl('zeroCrossEnable', gcbh);
      mask Display: disp(str)
  Out : Outport  VectorParamsAs1DForOutWhenUnconnected=off
  wires:
  dcm/1 -> Determinant of 3x3 Matrix/1(Matrix)
  Determinant of 3x3 Matrix/1(det(Matrix)) -> Bias/1
  Bias/1 -> Abs1/1
  Abs1/1 -> determinant does not equal 1/1(u)
  determinant does not equal 1/1(y) -> Out/1

== system viikate_rocket/Simple Variable Mass 6DOF/Calculate DCM & Euler Angles/Quaternions to Rotation Angles/Quat2DCM/Quaternion Normalize/Quaternion Modulus/Quaternion Norm ==
  q : Inport  Unit=1
  Demux : Demux
  Product{,1..3} (4 alike) : Product
  Sum : Sum  Inputs=4
  norm(q) : Outport  Unit=1  VectorParamsAs1DForOutWhenUnconnected=off
  wires:
  Demux/4 -> Product3/1, Product3/2
  Demux/3 -> Product2/1, Product2/2
  Demux/2 -> Product1/1, Product1/2
  Demux/1 -> Product/1, Product/2
  Product3/1 -> Sum/4
  Product2/1 -> Sum/3
  Product1/1 -> Sum/2
  Product/1 -> Sum/1
  Sum/1 -> norm(q)/1
  q/1 -> Demux/1

== system viikate_rocket/Simple Variable Mass 6DOF/Calculate DCM & Euler Angles/Quaternions to Rotation Angles/DCM2Ang/Validate DCM/If Warning//Error/Else If Not Orthogonal/Error ==
  In : Inport
  Action Port : ActionPort  InitializeStates=reset  ActionPortLabel=elseif(u1 == 3)
  Assertion : Assertion  AssertionFailFcn=sharedaeroassertmsg('validateDCM','notorthogonal','error')
  wires:
  In/1 -> Assertion/1

== system viikate_rocket/Simple Variable Mass 6DOF/Calculate DCM & Euler Angles/Quaternions to Rotation Angles/DCM2Ang/Validate DCM/If Warning//Error/Else If Not Orthogonal/None ==
  Action Port : ActionPort  ActionPortLabel=else

== system viikate_rocket/Simple Variable Mass 6DOF/Calculate DCM & Euler Angles/Quaternions to Rotation Angles/DCM2Ang/Validate DCM/If Warning//Error/Else If Not Orthogonal/Warning ==
  In : Inport
  Action Port : ActionPort  InitializeStates=reset  ActionPortLabel=if(u1 == 2)
  Assertion : Assertion  AssertionFailFcn=sharedaeroassertmsg('validateDCM','notorthogonal','warning')  StopWhenAssertionFail=off
  wires:
  In/1 -> Assertion/1

== system viikate_rocket/Simple Variable Mass 6DOF/Calculate DCM & Euler Angles/Quaternions to Rotation Angles/DCM2Ang/Validate DCM/If Warning//Error/If Not Proper/Error ==
  In : Inport
  Action Port : ActionPort  ActionPortLabel=elseif(u1 == 3)
  Assertion : Assertion  AssertionFailFcn=sharedaeroassertmsg('validateDCM','notproper','error')
  wires:
  In/1 -> Assertion/1

== system viikate_rocket/Simple Variable Mass 6DOF/Calculate DCM & Euler Angles/Quaternions to Rotation Angles/DCM2Ang/Validate DCM/If Warning//Error/If Not Proper/None ==
  Action Port : ActionPort  ActionPortLabel=else

== system viikate_rocket/Simple Variable Mass 6DOF/Calculate DCM & Euler Angles/Quaternions to Rotation Angles/DCM2Ang/Validate DCM/If Warning//Error/If Not Proper/Warning ==
  In : Inport
  Action Port : ActionPort  ActionPortLabel=if(u1 == 2)
  Assertion : Assertion  AssertionFailFcn=sharedaeroassertmsg('validateDCM','notproper','warning')  StopWhenAssertionFail=off
  wires:
  In/1 -> Assertion/1

== system viikate_rocket/Simple Variable Mass 6DOF/Calculate DCM & Euler Angles/Quaternions to Rotation Angles/DCM2Ang/Validate DCM/If Warning//Error/isNotOrthogonal/transpose*dcm ~= eye(3) ==
  u : Inport
  Compare : RelationalOperator  Operator=>  OutDataTypeStr=boolean
  Constant : Constant  DisableCoverage=on  Value=const  OutDataTypeStr=Inherit: Inherit via back propagation
  y : Outport
  wires:
  u/1 -> Compare/1
  Constant/1 -> Compare/2
  Compare/1 -> y/1

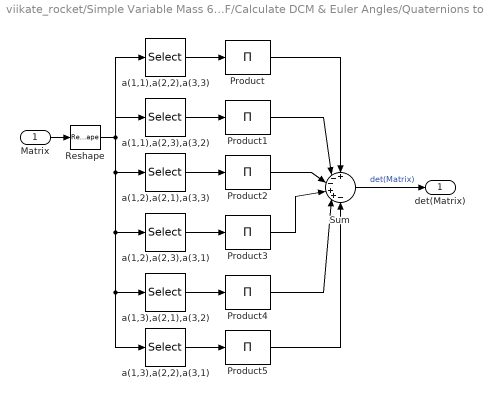
== system viikate_rocket/Simple Variable Mass 6DOF/Calculate DCM & Euler Angles/Quaternions to Rotation Angles/DCM2Ang/Validate DCM/If Warning//Error/isNotProper/Determinant of 3x3 Matrix ==
  Matrix : Inport  PortDimensions=[3 3]
  Product{,1..5} (6 alike) : Product  Inputs=1  SaturateOnIntegerOverflow=on  OutDataTypeStr=Inherit: Same as first input
  Reshape : Reshape  OutputDimensionality=Column vector (2-D)
  Sum : Sum  Inputs=+--++-  SaturateOnIntegerOverflow=on
  a(1,1),a(2,2),a(3,3) : Selector  InputPortWidth=9  IndexOptions=Index vector (dialog)  Indices=[1 5 9]  OutputSizes=1  RuntimeRangeChecks=off
  a(1,1),a(2,3),a(3,2) : Selector  InputPortWidth=9  IndexOptions=Index vector (dialog)  Indices=[1 6 8]  OutputSizes=1  RuntimeRangeChecks=off
  a(1,2),a(2,1),a(3,3) : Selector  InputPortWidth=9  IndexOptions=Index vector (dialog)  Indices=[2 4 9]  OutputSizes=1  RuntimeRangeChecks=off
  a(1,2),a(2,3),a(3,1) : Selector  InputPortWidth=9  IndexOptions=Index vector (dialog)  Indices=[3 4 8]  OutputSizes=1  RuntimeRangeChecks=off
  a(1,3),a(2,1),a(3,2) : Selector  InputPortWidth=9  IndexOptions=Index vector (dialog)  Indices=[2 6 7]  OutputSizes=1  RuntimeRangeChecks=off
  a(1,3),a(2,2),a(3,1) : Selector  InputPortWidth=9  IndexOptions=Index vector (dialog)  Indices=[3 5 7]  OutputSizes=1  RuntimeRangeChecks=off
  det(Matrix) : Outport  PortDimensions=1  VectorParamsAs1DForOutWhenUnconnected=off
  wires:
  Reshape/1 -> a(1,3),a(2,2),a(3,1)/1, a(1,3),a(2,1),a(3,2)/1, a(1,2),a(2,3),a(3,1)/1, a(1,2),a(2,1),a(3,3)/1, a(1,1),a(2,3),a(3,2)/1, a(1,1),a(2,2),a(3,3)/1
  Sum/1 -> det(Matrix)/1  "det(Matrix)"
  Matrix/1 -> Reshape/1
  Product5/1 -> Sum/6
  Product4/1 -> Sum/5
  Product3/1 -> Sum/4
  Product2/1 -> Sum/3
  Product1/1 -> Sum/2
  Product/1 -> Sum/1
  a(1,3),a(2,2),a(3,1)/1 -> Product5/1
  a(1,3),a(2,1),a(3,2)/1 -> Product4/1
  a(1,2),a(2,3),a(3,1)/1 -> Product3/1
  a(1,2),a(2,1),a(3,3)/1 -> Product2/1
  a(1,1),a(2,3),a(3,2)/1 -> Product1/1
  a(1,1),a(2,2),a(3,3)/1 -> Product/1
